simulink model "W08_SineSweep"  (R2024b)
settings: Solver=ode45  StartTime=0.0  StopTime=t_end  MaxStep=0.01  RelTol=1e-3
PreLoadFcn:
  | % W08_SineSweep 기본 파라미터 (모델을 열 때 자동 실행)
  | % 기본값은 질량-스프링-댐퍼, 입력 주파수 1 rad/s
  | defs = { 'A_in',1 ; 'w_in',1 ; 't_end',60 ;
  |          'numG',1 ; 'denG',[1 0.2 1] };
  | for ii = 1:size(defs,1)
  |     if ~evalin('base', sprintf('exist(''%s'',''var'')', defs{ii,1}))
  |         assignin('base', defs{ii,1}, defs{ii,2});
  |     end
  | end
  | clear defs ii
values from neighbouring files (symbols this model uses):
  A_in = 1    [W08_03_run_simulink.m]    (also in W08_04_slide_examples.m = 2; W08_05_rc_simulink.m)
  denG = [tau_1 1]    [W08_05_rc_simulink.m]
  numG = 1    [W08_05_rc_simulink.m]
  w_in = 1.0    (= 1)    [W08_03_run_simulink.m]
settings Model: Creator=admin  LastModifiedBy=admin

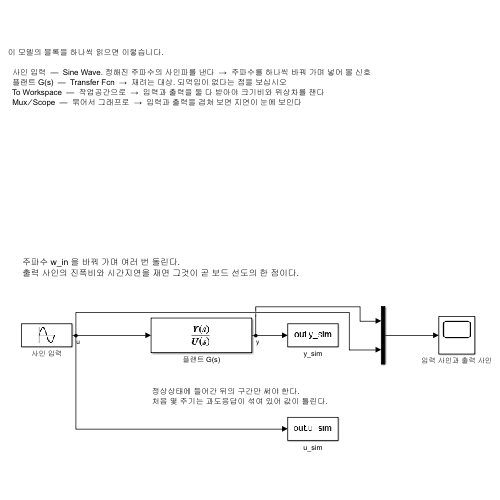
[thumbnail: Simulink's stored preview of the top-level diagram]
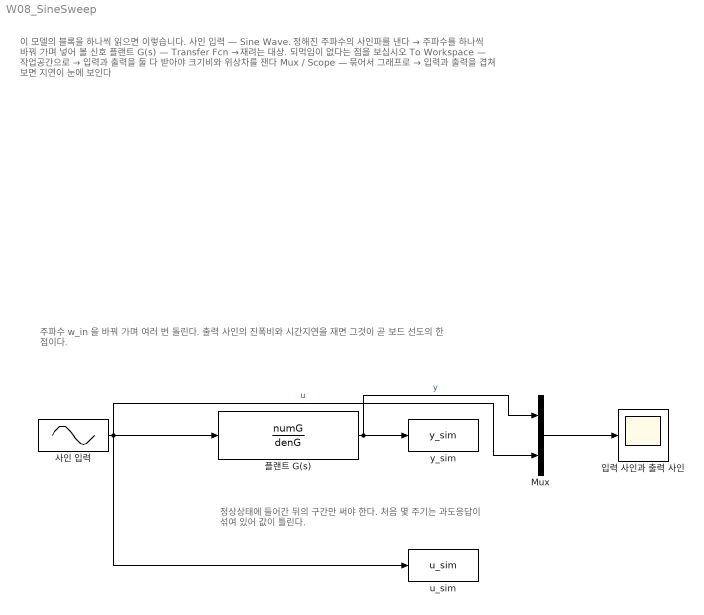
== system W08_SineSweep ==
  note: 주파수 w_in 을 바꿔 가며 여러 번 돌린다.
      | 출력 사인의 진폭비와 시간지연을 재면 그것이 곧 보드 선도의 한 점이다.
  note: 정상상태에 들어간 뒤의 구간만 써야 한다.
      | 처음 몇 주기는 과도응답이 섞여 있어 값이 틀린다.
  note: 이 모델의 블록을 하나씩 읽으면 이렇습니다.
      |
      |   사인 입력  —  Sine Wave. 정해진 주파수의 사인파를 낸다  →  주파수를 하나씩 바꿔 가며 넣어 볼 신호
      |   플랜트 G(s)  —  Transfer Fcn  →  재려는 대상. 되먹임이 없다는 점을 보십시오
      |   To Workspace  —  작업공간으로  →  입력과 출력을 둘 다 받아야 크기비와 위상차를 잰다
      |   Mux ∕ Scope  —  묶어서 그래프로  →  입력과 출력을 겹쳐 보면 지연이 눈에 보인다
  Mux : Mux  Inputs=2
  u_sim : ToWorkspace  VariableName=u_sim  SaveFormat=Timeseries  SampleTime=-1
  y_sim : ToWorkspace  VariableName=y_sim  SaveFormat=Timeseries  SampleTime=-1
  사인 입력 : Sin  Amplitude=A_in  Frequency=w_in  SampleTime=0
  입력 사인과 출력 사인 : Scope
  플랜트 G(s) : TransferFcn  Numerator=numG  Denominator=denG
  wires:
  사인 입력/1 -> 플랜트 G(s)/1, Mux/2, u_sim/1  "u"
  플랜트 G(s)/1 -> y_sim/1, Mux/1  "y"
  Mux/1 -> 입력 사인과 출력 사인/1
